simulink model "single_motor_fix_ob"  (R2025b)
settings: Solver=VariableStepAuto  StartTime=0.0  StopTime=10.0  RelTol=1e-3
values from neighbouring files (symbols this model uses):
  Dm = 1e-3    (= 0.001)    [motor_param.m]
  Jm = 0.1e-3    (= 0.0001)    [motor_param.m]
  Ld = 0.01    [motor_param.m]
  Lq = 0.02    [motor_param.m]
  p = 2    [motor_param.m]
  Phi = 0.1    [motor_param.m]
  Rs = 0.38    [motor_param.m]
libraries: fl_lib x10, nesl_utility x10, ee_lib x3, eeTransforms x2, simulink x1
settings Model: Creator=ZhiyongXu  LastModifiedBy=ZhiyongXu

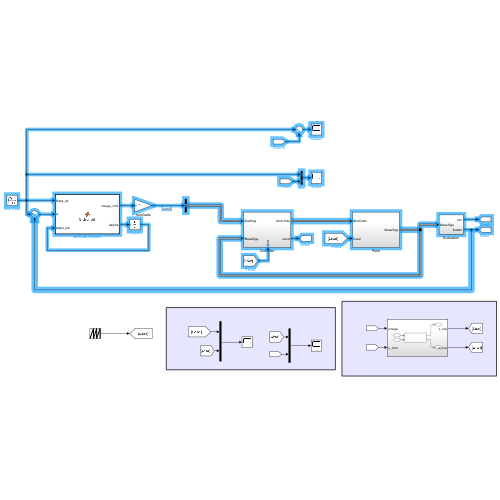
[thumbnail: Simulink's stored preview of the top-level diagram]
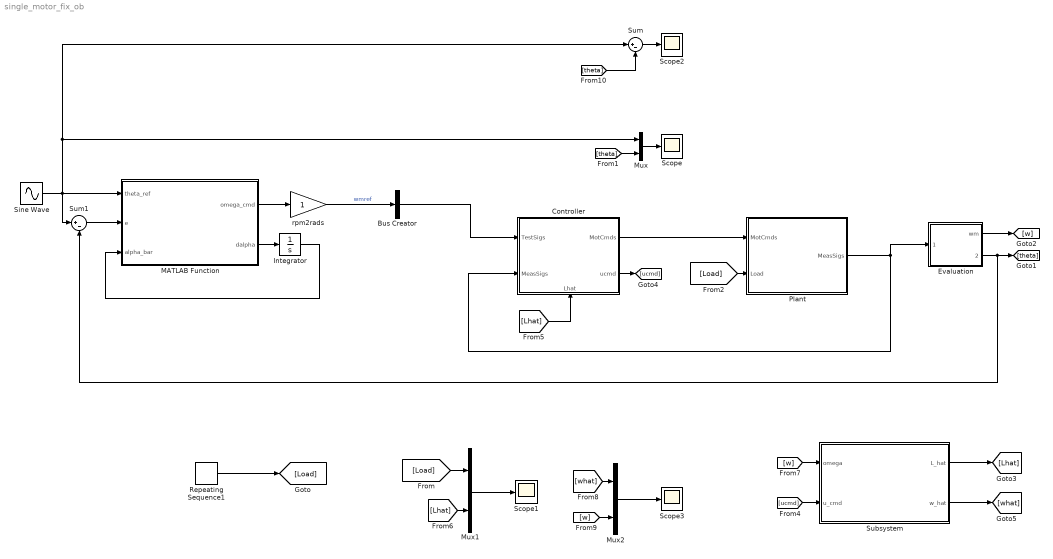
== system single_motor_fix_ob ==
  Bus Creator : BusCreator  Inputs=1
  Controller : Subsystem
      settings: PortSchema="{\"entries\":[{\"content\":{\"sides\":[{\"content\":{\"connectorIds\":[\"In1\",\"In2\"]},\"type\":\"ConnectorPlacement.EquallySpacedRectSide\",\"uuid\":\"9e2b7147-e799-4c99-9228-9f42ff49c31e\"},{\"content\":{\"connectorIds\":[\"Out1\",\"Out2\"],\"side\":\"RIGHT\"},\"type\":\"ConnectorPlacement.EquallySpacedRectSide\",\"uuid\":\"5daf7c61-761d-432c-b0c6-a04b6ede1655\"},{\"content\":{\"side\":\"TOP\"},\"type\":\"ConnectorPlacement.EquallySpacedRectSide\",\"uuid\":\"cb3e63cd-d58b-43da-aedb-4cfde167c947\"},{\"content\":{\"connectorIds\":[\"In3\"],\"side\":\"BOTTOM\"},\"type\":\"ConnectorPlacement.EquallySpacedRectSide\",\"uuid\":\"6a69f8ee-1dd9-44af-9de3-baa5c4959647\"}]},\"type\":\"ConnectorPlacement.EquallySpacedConnector\",\"uuid\":\"52e552b5-0aff-45e9-9ec7-cd907c785845\"}],\"packageUris\":[\"http://schema.mathworks.com/mf0/Connector/R2020b\"],\"version\":\"1.0\"}"
  Evaluation : Subsystem
  Integrator : Integrator
  MATLAB Function : MATLAB Function  TreatAsAtomicUnit=on
  Mux : Mux  Inputs=2
  Mux1 : Mux  Inputs=2
  Mux2 : Mux  Inputs=2
  Plant : Subsystem
  Repeating Sequence1 : simulink/Sources/Repeating Sequence  rep_seq_t=[0 5]  rep_seq_y=[-2 2]
  Scope{,1..3} (4 alike) : Scope
      Scope settings: ActiveDisplayYMinimum=-12.501085147532748  ActiveDisplayYMaximum=12.501085862817705
      Scope1 settings: ActiveDisplayYMinimum=-2.3570254189367765  ActiveDisplayYMaximum=4.7858750885523857  DataLoggingVariableName=ScopeData13
      Scope2 settings: ActiveDisplayYMinimum=-0.019188596634207  ActiveDisplayYMaximum=0.12297813424162181  DataLoggingVariableName=ScopeData3
      Scope3 settings: ActiveDisplayYMinimum=-76.914427455866786  ActiveDisplayYMaximum=97.497634288588515  DataLoggingVariableName=ScopeData14
  Sine Wave : Sin  Amplitude=10  SampleTime=0
  Subsystem : Subsystem
  Sum : Sum  Inputs=|+-
  Sum1 : Sum  Inputs=|+-
  rpm2rads : Gain
  wires:
  Mux/1 -> Scope/1
  Sum/1 -> Scope2/1
  Controller/2(ucmd) -> [ucmd]
  [what] -> Mux2/1
  Mux1/1 -> Scope1/1
  Mux2/1 -> Scope3/1
  rpm2rads/1 -> Bus Creator/1  "wmref"
  Bus Creator/1 -> Controller/1(TestSigs)
  Subsystem/1(L_hat) -> [Lhat]
  Controller/1(MotCmds) -> Plant/1(MotCmds)
  [w] -> Subsystem/1(omega)
  [Lhat] -> Controller/3(Lhat)
  Subsystem/2(w_hat) -> [what]
  [Load] -> Mux1/1
  Plant/1(MeasSigs) -> Controller/2(MeasSigs), Evaluation/1(MeasSigs)
  [ucmd] -> Subsystem/2(u_cmd)
  [w] -> Mux2/2
  Evaluation/1(wm) -> [w]
  [Lhat] -> Mux1/2
  Repeating Sequence1/1 -> [Load]
  [Load] -> Plant/2(Load)
  [theta] -> Mux/2
  [theta] -> Sum/2
  Evaluation/2(thetam) -> Sum1/2, [theta]
  Sine Wave/1 -> Mux/1, Sum/1, Sum1/1, MATLAB Function/1(theta_ref)
  MATLAB Function/1(omega_cmd) -> rpm2rads/1
  MATLAB Function/2(dalpha) -> Integrator/1
  Integrator/1 -> MATLAB Function/3(alpha_bar)
  Sum1/1 -> MATLAB Function/2(e)

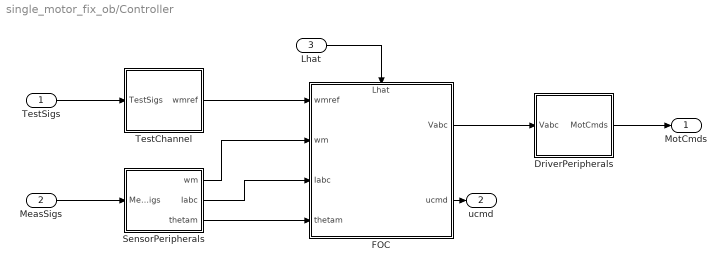
== system single_motor_fix_ob/Controller ==
  TestSigs : Inport
  MeasSigs : Inport  Port=2
  Lhat : Inport  Port=3
  DriverPeripherals : Subsystem
  FOC : Subsystem
      settings: PortSchema="{\"entries\":[{\"content\":{\"sides\":[{\"content\":{\"connectorIds\":[\"In1\",\"In2\",\"In3\",\"In4\"]},\"type\":\"ConnectorPlacement.EquallySpacedRectSide\",\"uuid\":\"766790a2-4c64-4515-982d-8e2c458e3cd3\"},{\"content\":{\"connectorIds\":[\"Out1\",\"Out2\"],\"side\":\"RIGHT\"},\"type\":\"ConnectorPlacement.EquallySpacedRectSide\",\"uuid\":\"84c791bf-b0b4-430e-add4-559453fc38c4\"},{\"content\":{\"connectorIds\":[\"In5\"],\"side\":\"TOP\"},\"type\":\"ConnectorPlacement.EquallySpacedRectSide\",\"uuid\":\"170d14ac-b1a9-4579-b469-c345e8cb6ac3\"}]},\"type\":\"ConnectorPlacement.EquallySpacedConnector\",\"uuid\":\"b234371d-3252-4452-947a-cf70bd43e9b7\"}],\"packageUris\":[\"http://schema.mathworks.com/mf0/Connector/R2020b\"],\"version\":\"1.0\"}"
  SensorPeripherals : Subsystem
  TestChannel : Subsystem
  MotCmds : Outport  VectorParamsAs1DForOutWhenUnconnected=off
  ucmd : Outport  Port=2
  wires:
  FOC/1(Vabc) -> DriverPeripherals/1(Vabc)
  DriverPeripherals/1(MotCmds) -> MotCmds/1
  TestSigs/1 -> TestChannel/1(TestSigs)
  TestChannel/1(wmref) -> FOC/1(wmref)
  MeasSigs/1 -> SensorPeripherals/1(MeasSigs)
  SensorPeripherals/1(wm) -> FOC/2(wm)
  SensorPeripherals/2(Iabc) -> FOC/3(Iabc)
  SensorPeripherals/3(thetam) -> FOC/4(thetam)
  FOC/2(ucmd) -> ucmd/1
  Lhat/1 -> FOC/5(Lhat)

== system single_motor_fix_ob/Evaluation ==
  MeasSigs : Inport
  Bus Selector1 : BusSelector  OutputSignals=wm,thetam
  wm : Outport
  thetam : Outport  Port=2
  wires:
  MeasSigs/1 -> Bus Selector1/1
  Bus Selector1/1 -> wm/1  "<wm>"
  Bus Selector1/2 -> thetam/1  "<thetam>"

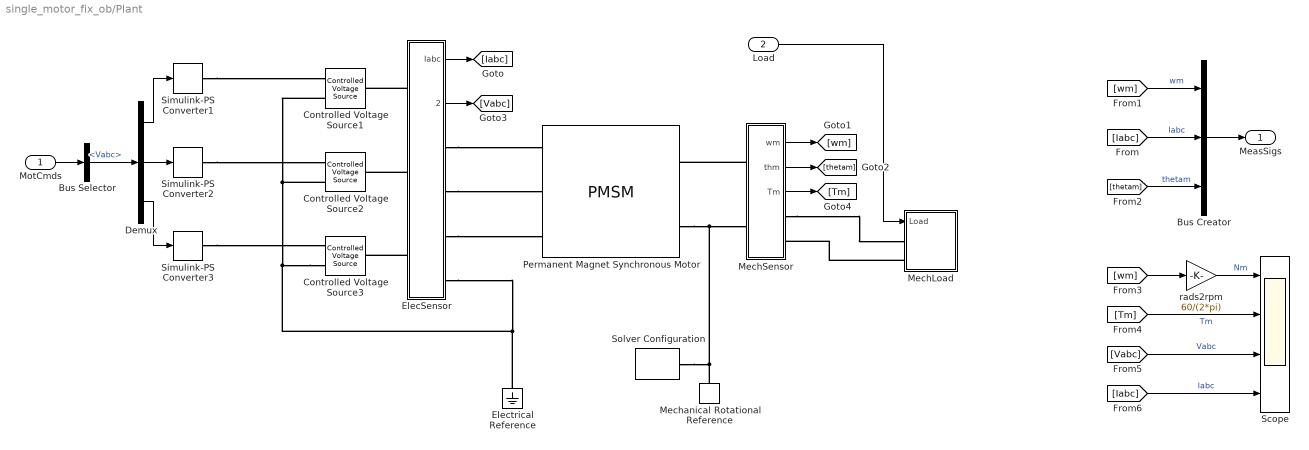
== system single_motor_fix_ob/Plant ==
  MotCmds : Inport
  Load : Inport  Port=2
  Bus Creator : BusCreator  Inputs=3
  Bus Selector : BusSelector  OutputSignals=Vabc
  Controlled Voltage Source1 : fl_lib/Electrical/Electrical Sources/Controlled Voltage Source
  Controlled Voltage Source2 : fl_lib/Electrical/Electrical Sources/Controlled Voltage Source
  Controlled Voltage Source3 : fl_lib/Electrical/Electrical Sources/Controlled Voltage Source
  Demux : Demux  Outputs=3
  ElecSensor : Subsystem
  Electrical Reference : fl_lib/Electrical/Electrical Elements/Electrical Reference
  MechLoad : Subsystem
  MechSensor : Subsystem
  Mechanical Rotational Reference : fl_lib/Mechanical/Rotational Elements/Mechanical Rotational Reference
  Permanent Magnet Synchronous Motor : ee_lib/Electromechanical/Permanent Magnet/PMSM  port_option=ee.enum.threePhasePort.expanded  winding_type=ee.enum.statorconnection.wye  machine_param=ee.enum.pmsm.parameterization.constant  nPolePairs=p  pmflux_param=1  pm_flux_linkage=Phi Wb  torque_constant=0.18 N*m/A  back_emf_constant=0.18 V/(rad/s)  stator_param=1  Ld=Ld H  Lq=Lq H  idVec=[-200, 0, 200] A  iqVec=[-200, 0, 200] A  LdMatrix=0.0002 * ones(3, 3) H  LqMatrix=0.0002 * ones(3, 3) H  PmMatrix=0.1 * ones(3, 3) Wb  ktMatrix=0.18 * ones(3, 3) N*m/A  keMatrix=0.18 * ones(3, 3) V/(rad/s)  L0=0 H  Ls=0.0002 H  Lm=-0.00002 H  Ms=0.00002 H  Rs=Rs Ohm  zero_sequence=ee.enum.park.zerosequence.exclude  axes_param=2  loss_param=ee.enum.ironloss.none  losses_oc=[0, 0, 0] W  losses_sc=[0, 0, 0] W  f_losses=60 Hz  Isc_losses=95 A  J=0 kg*m^2  lam=0 N*m/(rad/s)  i_d_specify=off  i_d_priority=None  i_d=0 A  i_d_nominal_specify=off  i_d_nominal_value=1  i_d_nominal_unit=A  i_q_specify=off  i_q_priority=None  i_q=0 A  i_q_nominal_specify=off  i_q_nominal_value=1  i_q_nominal_unit=A  torque_specify=off  torque_priority=None  torque=0 N*m  torque_nominal_specify=off  torque_nominal_value=1  torque_nominal_unit=N*m  angular_velocity_specify=on  angular_velocity_priority=High  angular_velocity=0 rpm  angular_velocity_nominal_specify=off  angular_velocity_nominal_value=1  angular_velocity_nominal_unit=rpm  angular_position_specify=off  angular_position_priority=High  angular_position=0 deg  angular_position_nominal_specify=off  angular_position_nominal_value=1  angular_position_nominal_unit=deg  alpha=3.93e-3 1/K  alpha_flux=-0.001 1/K  Tmeas=298.15 K  stator_thermal_mass=100 J/K  rotor_thermal_mass=200 J/K  Rm_percent_rotor=90  Rd_percent_rotor=30  temperatureA_specify=off  temperatureA_priority=High  temperatureA=25 degC  temperatureA_nominal_specify=off  temperatureA_nominal_value=1  temperatureA_nominal_unit=degC  temperatureB_specify=off  temperatureB_priority=High  temperatureB=25 degC  temperatureB_nominal_specify=off  temperatureB_nominal_value=1  temperatureB_nominal_unit=degC  temperatureC_specify=off  temperatureC_priority=High  temperatureC=25 degC  temperatureC_nominal_specify=off  temperatureC_nominal_value=1  temperatureC_nominal_unit=degC  temperatureR_specify=off  temperatureR_priority=High  temperatureR=25 degC  temperatureR_nominal_specify=off  temperatureR_nominal_value=1  temperatureR_nominal_unit=degC
      settings: InternalSimscapePortConfiguration="{\"Bottom\":[],\"Left\":[{\"id\":\"a\",\"label\":\"a\",\"type\":\"foundation.electrical.electrical\"},{\"id\":\"b\",\"label\":\"b\",\"type\":\"foundation.electrical.electrical\"},{\"id\":\"c\",\"label\":\"c\",\"type\":\"foundation.electrical.electrical\"}],\"Right\":[{\"id\":\"R\",\"label\":\"R\",\"type\":\"foundation.mechanical.rotational.rotational\"},{\"id\":\"C\",\"label\":\"C\",\"type\":\"foundation.mechanical.rotational.rotational\"}],\"Top\":[]}"
  Scope : Scope  NumInputPorts=4
      settings: ActiveDisplayYMinimum=-2500.2768341970282  ActiveDisplayYMaximum=2500.1048598569782
  Simulink-PS Converter1 : nesl_utility/Simulink-PS Converter  PhysicalDomain=network_engine_domain  SubClassName=ps_input  LeftPortType=input  RightPortType=output  PseudoPeriodic=off  Frequencies=[]  NoiseDistribution=none  NoiseParameters=[]  Unit=1  AffineConversion=off  FilteringAndDerivatives=provide  SimscapeFilterOrder=1  InputFilterTimeConstant=1e-6  UdotUserProvided=0
  Simulink-PS Converter2 : nesl_utility/Simulink-PS Converter  PhysicalDomain=network_engine_domain  SubClassName=ps_input  LeftPortType=input  RightPortType=output  PseudoPeriodic=off  Frequencies=[]  NoiseDistribution=none  NoiseParameters=[]  Unit=1  AffineConversion=off  FilteringAndDerivatives=provide  SimscapeFilterOrder=1  InputFilterTimeConstant=1e-6  UdotUserProvided=0
  Simulink-PS Converter3 : nesl_utility/Simulink-PS Converter  PhysicalDomain=network_engine_domain  SubClassName=ps_input  LeftPortType=input  RightPortType=output  PseudoPeriodic=off  Frequencies=[]  NoiseDistribution=none  NoiseParameters=[]  Unit=1  AffineConversion=off  FilteringAndDerivatives=provide  SimscapeFilterOrder=1  InputFilterTimeConstant=1e-6  UdotUserProvided=0
  Solver Configuration : nesl_utility/Solver Configuration  PhysicalDomain=network_engine_domain  SubClassName=solver  LeftPortType=input  RightPortType=generic  Tones=[]  Harmonics=[]  SimulateNoise=off  Profile=off  UseLocalSampling=off  EnableSwitchedLinearOptims=on  FrequencyDomain=off  UseCCode=off  RelTol=0.001  AbsTol=1e-06  MinStep=1e-09  ToWorkspace=off  RevertToSquareIcSolve=off  NumHomotopyIterations=100  PhasorMode=off  PhasorModeNumHarmonics=1  ConsistencySolver=NEWTON_XTOL_AFTER_FTOL  IndexReductionMethod=DerivativeReplacement  DoDC=off  ResidualTolerance=1e-09  ConsistencyTolSource=GLOBAL  ConsistencyAbsTol=0.001  ConsistencyRelTol=0.001  ConsistencyTolFactor=0.001  UseLocalSolver=off  LocalSolverChoice=NE_BACKWARD_EULER_ADVANCER  ResolveIndetEquations=on  FunctionEvalNumThread=1  LocalSolverSampleTime=0.001  DoFixedCost=off  MaxNonlinIter=3  MaxModeIter=2  ComputeImpulses=off  ImpulseIterations=2  LinearAlgebra=Sparse  LinearAlgebraNumThread=0  EquationFormulation=NE_TIME_EF  DelaysMemoryBudget=1024  AutomaticFiltering=on  FilteringTimeConstant=0.001  PartitionStorageMethod=AS_NEEDED  PartitionMemoryBudget=1024  PartitionMethod=FAST  MultibodyUseLocalSolver=off  MultibodyLocalSolverChoice=ODE1  MultibodyLocalSolverSampleTime=0.001
  rads2rpm : Gain  Gain=60/(2*pi)
  MeasSigs : Outport  VectorParamsAs1DForOutWhenUnconnected=off
  wires:
  ElecSensor/1(Iabc) -> [Iabc]
  ElecSensor/2(Vabc) -> [Vabc]
  Demux/2 -> Simulink-PS Converter2/1
  Demux/1 -> Simulink-PS Converter1/1
  Demux/3 -> Simulink-PS Converter3/1
  MechSensor/1(wm) -> [wm]
  MechSensor/2(thm) -> [thetam]
  MechSensor/3(Tm) -> [Tm]
  [wm] -> Bus Creator/1  "wm"
  [Iabc] -> Bus Creator/2  "Iabc"
  [thetam] -> Bus Creator/3  "thetam"
  Bus Creator/1 -> MeasSigs/1
  MotCmds/1 -> Bus Selector/1
  Bus Selector/1 -> Demux/1  "<Vabc>"
  [wm] -> rads2rpm/1
  rads2rpm/1 -> Scope/1  "Nm"
  [Tm] -> Scope/2  "Tm"
  [Vabc] -> Scope/3  "Vabc"
  [Iabc] -> Scope/4  "Iabc"
  Load/1 -> MechLoad/1(Load)
  connections:
  Simulink-PS Converter2/RConn1 -- Controlled Voltage Source2/RConn1
  Simulink-PS Converter3/RConn1 -- Controlled Voltage Source3/RConn1
  ElecSensor/RConn3 -- Permanent Magnet Synchronous Motor/LConn3
  ElecSensor/LConn2 -- Controlled Voltage Source2/LConn1
  Controlled Voltage Source3/RConn2 -- Controlled Voltage Source1/RConn2 -- Controlled Voltage Source2/RConn2 -- ElecSensor/RConn4 -- Electrical Reference/LConn1
  ElecSensor/RConn2 -- Permanent Magnet Synchronous Motor/LConn2
  ElecSensor/RConn1 -- Permanent Magnet Synchronous Motor/LConn1
  ElecSensor/LConn3 -- Controlled Voltage Source3/LConn1
  ElecSensor/LConn1 -- Controlled Voltage Source1/LConn1
  Simulink-PS Converter1/RConn1 -- Controlled Voltage Source1/RConn1
  Permanent Magnet Synchronous Motor/RConn2 -- Solver Configuration/RConn1 -- Mechanical Rotational Reference/LConn1 -- MechSensor/LConn2
  MechSensor/RConn1 -- MechLoad/LConn1
  MechLoad/LConn2 -- MechSensor/RConn2
  MechSensor/LConn1 -- Permanent Magnet Synchronous Motor/RConn1

== system single_motor_fix_ob/Subsystem ==
  omega : Inport
  u_cmd : Inport  Port=2
  observer : Subsystem
  L_hat : Outport
  w_hat : Outport  Port=2
  wires:
  omega/1 -> observer/1(omega)
  observer/1(L_hat) -> L_hat/1
  u_cmd/1 -> observer/2(u_cmd)
  observer/2(w_hat) -> w_hat/1

== system single_motor_fix_ob/Controller/DriverPeripherals ==
  Vabc : Inport
  Break Algebraic Loop : Subsystem
  Bus Creator : BusCreator  Inputs=1
  MotCmds : Outport  VectorParamsAs1DForOutWhenUnconnected=off
  wires:
  Vabc/1 -> Break Algebraic Loop/1(In1)
  Bus Creator/1 -> MotCmds/1
  Break Algebraic Loop/1(Out1) -> Bus Creator/1  "Vabc"

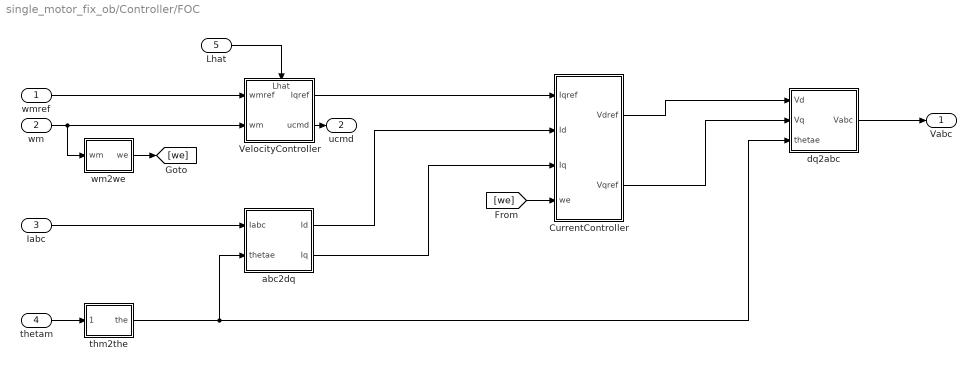
== system single_motor_fix_ob/Controller/FOC ==
  wmref : Inport
  wm : Inport  Port=2
  Iabc : Inport  Port=3
  thetam : Inport  Port=4
  Lhat : Inport  Port=5
  CurrentController : Subsystem
  VelocityController : Subsystem
      settings: PortSchema="{\"entries\":[{\"content\":{\"sides\":[{\"content\":{\"connectorIds\":[\"In1\",\"In2\"]},\"type\":\"ConnectorPlacement.EquallySpacedRectSide\",\"uuid\":\"9e2b7147-e799-4c99-9228-9f42ff49c31e\"},{\"content\":{\"connectorIds\":[\"Out1\",\"Out2\"],\"side\":\"RIGHT\"},\"type\":\"ConnectorPlacement.EquallySpacedRectSide\",\"uuid\":\"5daf7c61-761d-432c-b0c6-a04b6ede1655\"},{\"content\":{\"connectorIds\":[\"In3\"],\"side\":\"TOP\"},\"type\":\"ConnectorPlacement.EquallySpacedRectSide\",\"uuid\":\"cb3e63cd-d58b-43da-aedb-4cfde167c947\"}]},\"type\":\"ConnectorPlacement.EquallySpacedConnector\",\"uuid\":\"52e552b5-0aff-45e9-9ec7-cd907c785845\"}],\"packageUris\":[\"http://schema.mathworks.com/mf0/Connector/R2020b\"],\"version\":\"1.0\"}"
  abc2dq : Subsystem
  dq2abc : Subsystem
  thm2the : Subsystem
  wm2we : Subsystem
  Vabc : Outport  VectorParamsAs1DForOutWhenUnconnected=off
  ucmd : Outport  Port=2
  wires:
  abc2dq/2(Iq) -> CurrentController/3(Iq)
  wmref/1 -> VelocityController/1(wmref)
  abc2dq/1(Id) -> CurrentController/2(Id)
  Iabc/1 -> abc2dq/1(Iabc)
  CurrentController/1(Vdref) -> dq2abc/1(Vd)
  CurrentController/2(Vqref) -> dq2abc/2(Vq)
  [we] -> CurrentController/4(we)
  wm/1 -> VelocityController/2(wm), wm2we/1(wm)
  dq2abc/1(Vabc) -> Vabc/1
  VelocityController/1(Iqref) -> CurrentController/1(Iqref)
  thm2the/1(the) -> abc2dq/2(thetae), dq2abc/3(thetae)
  thetam/1 -> thm2the/1(thm)
  wm2we/1(we) -> [we]
  VelocityController/2(ucmd) -> ucmd/1
  Lhat/1 -> VelocityController/3(Lhat)

== system single_motor_fix_ob/Controller/SensorPeripherals ==
  MeasSigs : Inport
  Bus Selector : BusSelector  OutputSignals=wm,Iabc,thetam
  wm : Outport  VectorParamsAs1DForOutWhenUnconnected=off
  Iabc : Outport  Port=2  VectorParamsAs1DForOutWhenUnconnected=off
  thetam : Outport  Port=3  VectorParamsAs1DForOutWhenUnconnected=off
  wires:
  MeasSigs/1 -> Bus Selector/1
  Bus Selector/2 -> Iabc/1  "<Iabc>"
  Bus Selector/1 -> wm/1  "<wm>"
  Bus Selector/3 -> thetam/1  "<thetam>"

== system single_motor_fix_ob/Controller/TestChannel ==
  TestSigs : Inport
  Bus Selector : BusSelector  OutputSignals=wmref
  wmref : Outport  VectorParamsAs1DForOutWhenUnconnected=off
  wires:
  TestSigs/1 -> Bus Selector/1
  Bus Selector/1 -> wmref/1  "<wmref>"

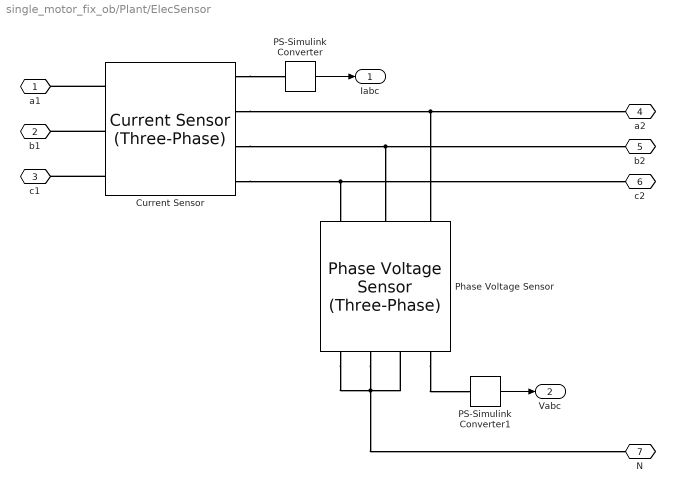
== system single_motor_fix_ob/Plant/ElecSensor ==
  Current Sensor : ee_lib/Sensors & Transducers/Current Sensor (Three-Phase)
      settings: InternalSimscapePortConfiguration="{\"Bottom\":[],\"Left\":[{\"id\":\"a1\",\"label\":\"a1\",\"type\":\"foundation.electrical.electrical\"},{\"id\":\"b1\",\"label\":\"b1\",\"type\":\"foundation.electrical.electrical\"},{\"id\":\"c1\",\"label\":\"c1\",\"type\":\"foundation.electrical.electrical\"}],\"Right\":[{\"id\":\"I_output\",\"label\":\"I\",\"type\":\"output\"},{\"id\":\"a2\",\"label\":\"a2\",\"type\":\"foundation.electrical.electrical\"},{\"id\":\"b2\",\"label\":\"b2\",\"type\":\"foundation.electrical.electrical\"},{\"id\":\"c2\",\"label\":\"c2\",\"type\":\"foundation.electrical.electrical\"}],\"Top\":[]}"
  PS-Simulink Converter : nesl_utility/PS-Simulink Converter  PhysicalDomain=network_engine_domain  SubClassName=ps_output  LeftPortType=input  RightPortType=output  PseudoPeriodic=off  Frequencies=[]  VectorFormat=1-D array  Unit=1  AffineConversion=off
  PS-Simulink Converter1 : nesl_utility/PS-Simulink Converter  PhysicalDomain=network_engine_domain  SubClassName=ps_output  LeftPortType=input  RightPortType=output  PseudoPeriodic=off  Frequencies=[]  VectorFormat=1-D array  Unit=1  AffineConversion=off
  Phase Voltage Sensor : ee_lib/Sensors & Transducers/Phase Voltage Sensor (Three-Phase)
      settings: InternalSimscapePortConfiguration="{\"Bottom\":[],\"Left\":[{\"id\":\"a1\",\"label\":\"a1\",\"type\":\"foundation.electrical.electrical\"},{\"id\":\"b1\",\"label\":\"b1\",\"type\":\"foundation.electrical.electrical\"},{\"id\":\"c1\",\"label\":\"c1\",\"type\":\"foundation.electrical.electrical\"}],\"Right\":[{\"id\":\"V_output\",\"label\":\"V\",\"type\":\"output\"},{\"id\":\"a2\",\"label\":\"a2\",\"type\":\"foundation.electrical.electrical\"},{\"id\":\"b2\",\"label\":\"b2\",\"type\":\"foundation.electrical.electrical\"},{\"id\":\"c2\",\"label\":\"c2\",\"type\":\"foundation.electrical.electrical\"}],\"Top\":[]}"
  a1 : PMIOPort  Side=Left
  b1 : PMIOPort  Port=2  Side=Left
  c1 : PMIOPort  Port=3  Side=Left
  a2 : PMIOPort  Port=4  Side=Right
  b2 : PMIOPort  Port=5  Side=Right
  c2 : PMIOPort  Port=6  Side=Right
  N : PMIOPort  Port=7  Side=Right
  Iabc : Outport  VectorParamsAs1DForOutWhenUnconnected=off
  Vabc : Outport  Port=2  VectorParamsAs1DForOutWhenUnconnected=off
  wires:
  PS-Simulink Converter/1 -> Iabc/1
  PS-Simulink Converter1/1 -> Vabc/1
  connections:
  Current Sensor/LConn1 -- a1/RConn1
  Current Sensor/LConn2 -- b1/RConn1
  Current Sensor/LConn3 -- c1/RConn1
  Current Sensor/RConn1 -- PS-Simulink Converter/LConn1
  Phase Voltage Sensor/RConn1 -- PS-Simulink Converter1/LConn1
  Current Sensor/RConn2 -- a2/RConn1 -- Phase Voltage Sensor/LConn1
  Current Sensor/RConn3 -- b2/RConn1 -- Phase Voltage Sensor/LConn2
  Current Sensor/RConn4 -- c2/RConn1 -- Phase Voltage Sensor/LConn3
  Phase Voltage Sensor/RConn4 -- N/RConn1 -- Phase Voltage Sensor/RConn3 -- Phase Voltage Sensor/RConn2

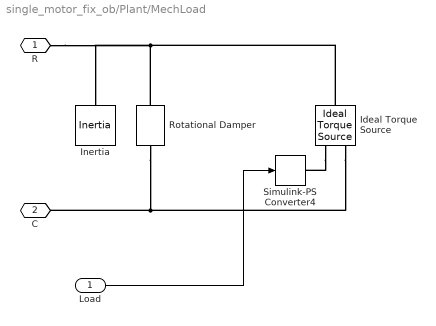
== system single_motor_fix_ob/Plant/MechLoad ==
  Load : Inport
  Ideal Torque Source : fl_lib/Mechanical/Mechanical Sources/Ideal Torque Source
  Inertia : fl_lib/Mechanical/Rotational Elements/Inertia  inertia=Jm kg*m^2  num_ports=foundation.enum.numPorts2.one  w_specify=on  w_priority=High  w=0 rpm  w_nominal_specify=off  w_nominal_value=1  w_nominal_unit=rad/s  t_specify=off  t_priority=None  t=0 N*m  t_nominal_specify=off  t_nominal_value=1  t_nominal_unit=N*m
  Rotational Damper : fl_lib/Mechanical/Rotational Elements/Rotational Damper  D=Dm N*m/(rad/s)  w_specify=off  w_priority=None  w=0 rad/s  w_nominal_specify=off  w_nominal_value=1  w_nominal_unit=rad/s  t_specify=off  t_priority=None  t=0 N*m  t_nominal_specify=off  t_nominal_value=1  t_nominal_unit=N*m
  Simulink-PS Converter4 : nesl_utility/Simulink-PS Converter  PhysicalDomain=network_engine_domain  SubClassName=ps_input  LeftPortType=input  RightPortType=output  PseudoPeriodic=off  Frequencies=[]  NoiseDistribution=none  NoiseParameters=[]  Unit=1  AffineConversion=off  FilteringAndDerivatives=provide  SimscapeFilterOrder=1  InputFilterTimeConstant=0.001  UdotUserProvided=0
  R : PMIOPort  Side=Left
  C : PMIOPort  Port=2  Side=Left
  wires:
  Load/1 -> Simulink-PS Converter4/1
  connections:
  Ideal Torque Source/RConn1 -- Simulink-PS Converter4/RConn1
  Rotational Damper/RConn1 -- Ideal Torque Source/RConn2 -- C/RConn1
  Rotational Damper/LConn1 -- Ideal Torque Source/LConn1 -- R/RConn1 -- Inertia/LConn1

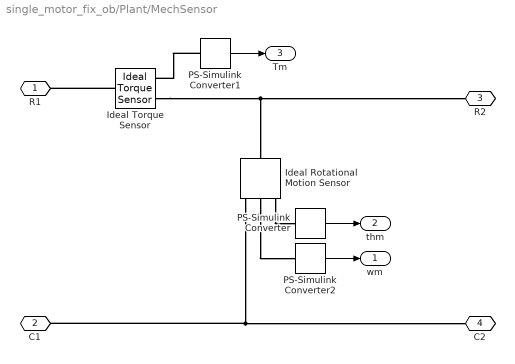
== system single_motor_fix_ob/Plant/MechSensor ==
  Ideal Rotational Motion Sensor : fl_lib/Mechanical/Mechanical Sensors/Ideal Rotational Motion Sensor  reference=foundation.enum.MeasurementReference.difference  acceleration_port=false  velocity_port=true  position_port=true  wrap_angle=simscape.enum.onoff.off  offset=0 rad
  Ideal Torque Sensor : fl_lib/Mechanical/Mechanical Sensors/Ideal Torque Sensor
  PS-Simulink Converter : nesl_utility/PS-Simulink Converter  PhysicalDomain=network_engine_domain  SubClassName=ps_output  LeftPortType=input  RightPortType=output  PseudoPeriodic=off  Frequencies=[]  VectorFormat=1-D array  Unit=1  AffineConversion=off
  PS-Simulink Converter1 : nesl_utility/PS-Simulink Converter  PhysicalDomain=network_engine_domain  SubClassName=ps_output  LeftPortType=input  RightPortType=output  PseudoPeriodic=off  Frequencies=[]  VectorFormat=1-D array  Unit=1  AffineConversion=off
  PS-Simulink Converter2 : nesl_utility/PS-Simulink Converter  PhysicalDomain=network_engine_domain  SubClassName=ps_output  LeftPortType=input  RightPortType=output  PseudoPeriodic=off  Frequencies=[]  VectorFormat=1-D array  Unit=1  AffineConversion=off
  R1 : PMIOPort  Side=Left
  C1 : PMIOPort  Port=2  Side=Left
  R2 : PMIOPort  Port=3  Side=Right
  C2 : PMIOPort  Port=4  Side=Right
  wm : Outport  VectorParamsAs1DForOutWhenUnconnected=off
  thm : Outport  Port=2  VectorParamsAs1DForOutWhenUnconnected=off
  Tm : Outport  Port=3  VectorParamsAs1DForOutWhenUnconnected=off
  wires:
  PS-Simulink Converter/1 -> thm/1
  PS-Simulink Converter1/1 -> Tm/1
  PS-Simulink Converter2/1 -> wm/1
  connections:
  Ideal Rotational Motion Sensor/RConn3 -- PS-Simulink Converter/LConn1
  Ideal Rotational Motion Sensor/RConn1 -- C2/RConn1 -- C1/RConn1
  Ideal Torque Sensor/LConn1 -- R1/RConn1
  Ideal Torque Sensor/RConn1 -- R2/RConn1 -- Ideal Rotational Motion Sensor/LConn1
  PS-Simulink Converter1/LConn1 -- Ideal Torque Sensor/RConn2
  Ideal Rotational Motion Sensor/RConn2 -- PS-Simulink Converter2/LConn1

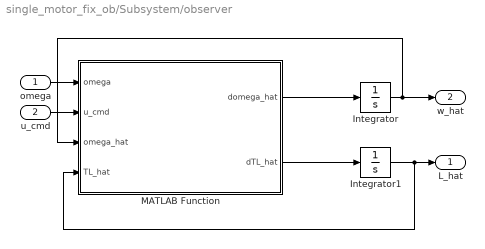
== system single_motor_fix_ob/Subsystem/observer ==
  omega : Inport
  u_cmd : Inport  Port=2
  Integrator : Integrator
  Integrator1 : Integrator
  MATLAB Function : MATLAB Function  TreatAsAtomicUnit=on
  L_hat : Outport
  w_hat : Outport  Port=2
  wires:
  MATLAB Function/1(domega_hat) -> Integrator/1
  MATLAB Function/2(dTL_hat) -> Integrator1/1
  Integrator/1 -> w_hat/1, MATLAB Function/3(omega_hat)
  Integrator1/1 -> L_hat/1, MATLAB Function/4(TL_hat)
  omega/1 -> MATLAB Function/1(omega)
  u_cmd/1 -> MATLAB Function/2(u_cmd)

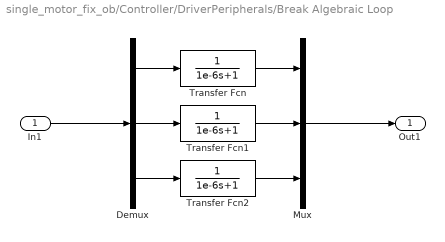
== system single_motor_fix_ob/Controller/DriverPeripherals/Break Algebraic Loop ==
  In1 : Inport
  Demux : Demux  Outputs=3
  Mux : Mux  Inputs=3
  Transfer Fcn : TransferFcn  Denominator=[1e-6 1]
  Transfer Fcn1 : TransferFcn  Denominator=[1e-6 1]
  Transfer Fcn2 : TransferFcn  Denominator=[1e-6 1]
  Out1 : Outport
  wires:
  In1/1 -> Demux/1
  Demux/1 -> Transfer Fcn/1
  Transfer Fcn/1 -> Mux/1
  Demux/2 -> Transfer Fcn1/1
  Transfer Fcn1/1 -> Mux/2
  Demux/3 -> Transfer Fcn2/1
  Transfer Fcn2/1 -> Mux/3
  Mux/1 -> Out1/1

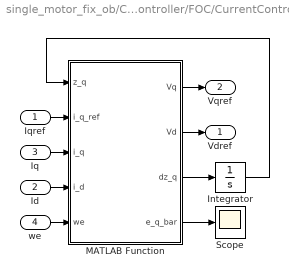
== system single_motor_fix_ob/Controller/FOC/CurrentController ==
  Iqref : Inport
  Id : Inport  Port=2
  Iq : Inport  Port=3
  we : Inport  Port=4
  Integrator : Integrator
  MATLAB Function : MATLAB Function  TreatAsAtomicUnit=on
  Scope : Scope
      settings: ActiveDisplayYMinimum=-0.021972241997855933  ActiveDisplayYMaximum=0.011100987286103392  DataLoggingVariableName=ScopeData15
  Vdref : Outport  VectorParamsAs1DForOutWhenUnconnected=off
  Vqref : Outport  Port=2  VectorParamsAs1DForOutWhenUnconnected=off
  wires:
  Integrator/1 -> MATLAB Function/1(z_q)
  MATLAB Function/3(dz_q) -> Integrator/1
  MATLAB Function/4(e_q_bar) -> Scope/1
  MATLAB Function/1(Vq) -> Vqref/1
  MATLAB Function/2(Vd) -> Vdref/1
  we/1 -> MATLAB Function/5(we)
  Iqref/1 -> MATLAB Function/2(i_q_ref)
  Id/1 -> MATLAB Function/4(i_d)
  Iq/1 -> MATLAB Function/3(i_q)

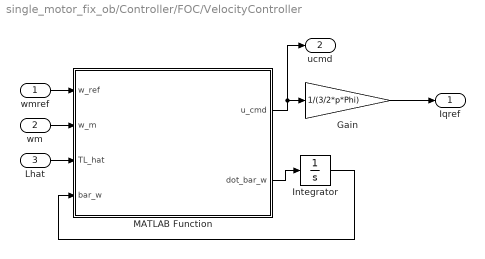
== system single_motor_fix_ob/Controller/FOC/VelocityController ==
  wmref : Inport
  wm : Inport  Port=2
  Lhat : Inport  Port=3
  Gain : Gain  Gain=1/(3/2*p*Phi)
  Integrator : Integrator
  MATLAB Function : MATLAB Function  TreatAsAtomicUnit=on
  Iqref : Outport  VectorParamsAs1DForOutWhenUnconnected=off
  ucmd : Outport  Port=2
  wires:
  Gain/1 -> Iqref/1
  MATLAB Function/1(u_cmd) -> ucmd/1, Gain/1
  MATLAB Function/2(dot_bar_w) -> Integrator/1
  Integrator/1 -> MATLAB Function/4(bar_w)
  wmref/1 -> MATLAB Function/1(w_ref)
  wm/1 -> MATLAB Function/2(w_m)
  Lhat/1 -> MATLAB Function/3(TL_hat)

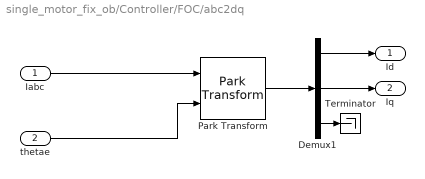
== system single_motor_fix_ob/Controller/FOC/abc2dq ==
  Iabc : Inport
  thetae : Inport  Port=2
  Demux1 : Demux  Outputs=3
  Park Transform : eeTransforms/Park Transform  AxisAlignment=D-axis  PowerInvariant=off
  Terminator : Terminator
  Id : Outport  VectorParamsAs1DForOutWhenUnconnected=off
  Iq : Outport  Port=2  VectorParamsAs1DForOutWhenUnconnected=off
  wires:
  Iabc/1 -> Park Transform/1
  thetae/1 -> Park Transform/2
  Demux1/3 -> Terminator/1
  Park Transform/1 -> Demux1/1
  Demux1/1 -> Id/1
  Demux1/2 -> Iq/1

== system single_motor_fix_ob/Controller/FOC/dq2abc ==
  Vd : Inport
  Vq : Inport  Port=2
  thetae : Inport  Port=3
  Constant : Constant  Value=0
  Inverse Park Transform : eeTransforms/Inverse Park Transform  AxisAlignment=D-axis  PowerInvariant=off
  Mux : Mux  Inputs=3
  Vabc : Outport  VectorParamsAs1DForOutWhenUnconnected=off
  wires:
  thetae/1 -> Inverse Park Transform/2
  Constant/1 -> Mux/3
  Mux/1 -> Inverse Park Transform/1
  Vd/1 -> Mux/1
  Inverse Park Transform/1 -> Vabc/1
  Vq/1 -> Mux/2

== system single_motor_fix_ob/Controller/FOC/thm2the ==
  thm : Inport
  Constant : Constant  Value=2*pi
  Mod : Math  Operator=mod  SignedPower=on
  PolePairs : Gain  Gain=p
  the : Outport  VectorParamsAs1DForOutWhenUnconnected=off
  wires:
  Constant/1 -> Mod/2
  PolePairs/1 -> Mod/1
  Mod/1 -> the/1
  thm/1 -> PolePairs/1

== system single_motor_fix_ob/Controller/FOC/wm2we ==
  wm : Inport
  PolePairs : Gain  Gain=p
  we : Outport  VectorParamsAs1DForOutWhenUnconnected=off
  wires:
  wm/1 -> PolePairs/1
  PolePairs/1 -> we/1

== matlab function single_motor_fix_ob/MATLAB Function ==
  data: theta_ref input; omega_cmd output; dalpha output; e input; alpha_bar input
function [omega_cmd, dalpha] = ft_dsc_ctrl(theta_ref, e, alpha_bar)
%#codegen
% 固定时间动态面 + 固定时间控制器
% 本块只算导数 dalpha 与控制量；alpha_bar 由外部 Integrator 积分

% ---------- 固定时间动态面参数 ----------
tau  = 0.005;
kf1  = 30;   pf1 = 0.5;
kf2  = 15;   pf2 = 1.5;

% ---------- 控制器参数 ----------
k1 = 5;  p1 = 0.5;
k2 =  5;  p2 = 1.5;

sig = @(v,p) (abs(v)^p) * sign(v);

% ---------- 动态面滤波器：只输出导数 ----------
delta  = alpha_bar - theta_ref;
dalpha = -( kf1*sig(delta,pf1) + kf2*sig(delta,pf2) ) / tau;

% ---------- om_ref 的估计 = alpha_bar 的导数 ----------
om_ref_hat = dalpha;

% ---------- 控制律 ----------
u = om_ref_hat + k1*sig(e,p1) + k2*sig(e,p2);

% ---------- ±50 饱和 ----------
omega_cmd = min(max(u, -50), 50);

end

== matlab function single_motor_fix_ob/Controller/FOC/CurrentController/MATLAB Function ==
  data: z_q input; Vq output; i_q_ref input; i_q input; i_d input; we input; Vd output; dz_q output; e_q_bar output; Rs parameter; Ld parameter; Lq parameter; Phi parameter
function [Vq, Vd, dz_q, e_q_bar] = smc_ctrl(z_q, i_q_ref, i_q, i_d, we, Rs, Ld, Lq, Phi)
%#codegen
% ============================================================
%  PMSM 超螺旋滑模电流控制器
%  Rs, Ld, Lq, Phi, p 及滑模增益均由 Parameter 作用域提供
% ============================================================

%% ---------- 滑模参数 (仍然写死, 因为它们只属于控制器) ----------
r1  = 0.5;   r2  = 1.5;
rho1 = 0.5;  rho2 = 1.5;

k_q1 = -5000;  k_q2 = -4000;
k_d1 = -5000;  k_d2 = -4000;

lam_q1 = 50;   lam_q2 = 50;

%% ---------- 滑模面 ----------
e_q_bar = i_q - z_q;

%% ---------- 迭代部分的导数 (积分交给 Simulink) ----------
e_z  = z_q - i_q_ref;
dz_q = -lam_q1 * sig(e_z, rho1) - lam_q2 * sig(e_z, rho2);

%% ---------- u_q (非迭代) ----------
Vq = Lq * ( dz_q ...
             + k_q1 * sig(e_q_bar, r1) ...
             + k_q2 * sig(e_q_bar, r2) ) ...
      + Rs * z_q ...
      + Ld * we * i_d ...
      + we * Phi ;

%% ---------- u_d (非迭代) ----------
Vd = Ld * ( k_d1 * sig(i_d, r1) ...
             + k_d2 * sig(i_d, r2) ) ...
      + Rs * i_d ...
      + Lq * we * i_q;

end

function y = sig(x, r)
    y = abs(x)^r * sign(x);
end

== matlab function single_motor_fix_ob/Subsystem/observer/MATLAB Function ==
  data: omega input; domega_hat output; u_cmd input; omega_hat input; TL_hat input; dTL_hat output; Jm parameter; Dm parameter
function [domega_hat, dTL_hat] = ftdop(omega, u_cmd, omega_hat, TL_hat, Jm, Dm)
%#codegen

%% ---------------- 观测器参数 ----------------
p1 = 0.6;
p2 = 1.4;

% k1 = 2.0;
% k2 = 2.0;
% k3 = 5.0;
% k4 = 30.0;
% k5 = 20.0;
% k6 = 20.0;


k1 = 20;    % 原 2
k2 = 20;    % 原 2
k3 = 50;    % 原 5

k4 = 100;   % 原 30
k5 = 100;   % 原 20
k6 = 80;   % 原 20
%% ---------------- 观测器计算 ----------------
eps = omega - omega_hat;

e_p1   = spow(eps, p1);
e_p2   = spow(eps, p2);
e_2p1m = spow(eps, 2*p1-1);
e_2p2m = spow(eps, 2*p2-1);

domega_hat = (u_cmd + TL_hat - Dm*omega_hat ...
              + k1*e_p1 + k2*e_p2 + k3*eps) / Jm;

% 注意：这里三个负号是修正后的关键
dTL_hat = k4*e_2p1m + k5*e_2p2m + k6*eps;
end

function y = spow(x, p)
absx = abs(x);
absx = max(absx, 1e-8);
y = sign(x) .* absx.^p;
y(x == 0) = 0;
end

== matlab function single_motor_fix_ob/Controller/FOC/VelocityController/MATLAB Function ==
  data: w_ref input; u_cmd output; w_m input; TL_hat input; bar_w input; dot_bar_w output; Jm parameter; Dm parameter
function [u_cmd, dot_bar_w] = FixedTimeController(w_ref, w_m, TL_hat, bar_w, Jm, Dm)

    % ---- 固定时间滤波器参数 ----
    lambda1  = 8;
    lambda2  = 8;
    lambda3  = 10;
    tau      = 0.5;
    vartheta = 1.5;

    % ---- 内环固定时间反馈参数 ----
    k_w = 8;
    k1  = 6;
    k2  = 6;

    pow_func = @(x, gamma) abs(x)^gamma * sign(x);

    % ---- 公式(117) 滤波器 ----
    e_w = bar_w - w_ref;
    dot_bar_w = (1/tau) * ( -lambda1 * pow_func(e_w, 0.5) ...
                            -lambda2 * pow_func(e_w, vartheta) ...
                            -lambda3 * e_w );

    % ---- 公式(121) 动态面偏差 ----
    s = w_m - bar_w;

    % ---- 公式(122) 内环力矩指令 ----
    feedforward = Jm * dot_bar_w + Dm * bar_w - TL_hat;
    feedback    = -k_w * s ...
                  - k1 * pow_func(s, 0.5) ...
                  - k2 * pow_func(s, vartheta);

    u_cmd = feedforward + feedback;
end
